simulink model "Sistemap3"  (R2026a)
settings: Solver=ode15s  StopTime=10  MaxStep=1E-2
libraries: fl_lib x14, nesl_utility x8, slpidlib x1
settings Model: Creator=Admin  LastModifiedBy=HP
settings DataIOCC: TimeSaveName=t
settings DebuggingCC: ArtificialAlgebraicLoopMsg=none  MaxConsecutiveZCsMsg=none

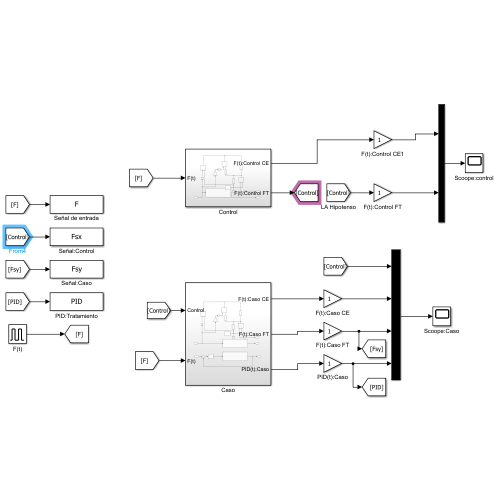
[thumbnail: Simulink's stored preview of the top-level diagram]
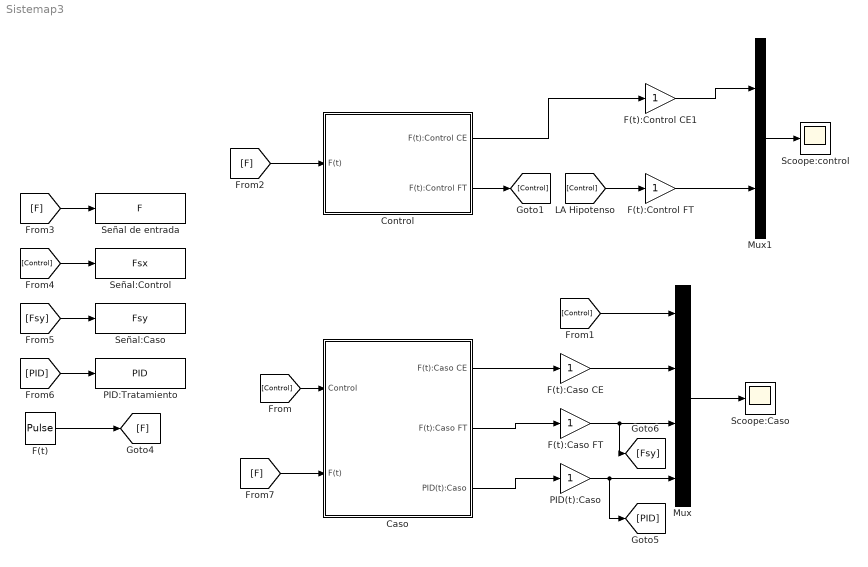
== system Sistemap3 ==
  Caso : Subsystem
  Control : Subsystem
  "F(t) " : DiscretePulseGenerator  PulseType=Time based  Period=10  PulseWidth=10  PhaseDelay=1
  F(t):Caso CE : Gain
  F(t):Caso FT : Gain
  F(t):Control CE1 : Gain
  F(t):Control FT : Gain
  Mux : Mux
  Mux1 : Mux  Inputs=2
  PID(t):Caso : Gain
  PID:Tratamiento : ToWorkspace  VariableName=PID  SampleTime=-1
  Scoope:Caso : Scope
      settings: TimeSpan=10  ActiveDisplayYMinimum=-0.21660297738034551  ActiveDisplayYMaximum=1.0433970226196547
  Scoope:control : Scope
      settings: ActiveDisplayYMinimum=-0.48996250674145203  ActiveDisplayYMaximum=1.2740374932585483
  Señal de entrada : ToWorkspace  VariableName=F  SampleTime=-1
  Señal:Caso : ToWorkspace  VariableName=Fsy  SampleTime=-1
  Señal:Control : ToWorkspace  VariableName=Fsx  SampleTime=-1
  wires:
  [Control] -> Caso/1(Control)
  [Control] -> Mux/1
  Mux/1 -> Scoope:Caso/1
  F(t):Caso CE/1 -> Mux/2
  F(t):Caso FT/1 -> [Fsy], Mux/3
  PID(t):Caso/1 -> [PID], Mux/4
  [F] -> Control/1(F(t))
  Mux1/1 -> Scoope:control/1
  Control/2(F(t):Control FT) -> [Control]
  [F] -> Señal de entrada/1
  [Control] -> Señal:Control/1
  [Fsy] -> Señal:Caso/1
  [PID] -> PID:Tratamiento/1
  "F(t) "/1 -> [F]
  [F] -> Caso/2(F(t))
  Caso/1(F(t):Caso CE) -> F(t):Caso CE/1
  Caso/2(F(t):Caso FT) -> F(t):Caso FT/1
  Caso/3(PID(t):Caso) -> PID(t):Caso/1
  [Control] -> F(t):Control FT/1
  F(t):Control FT/1 -> Mux1/2
  Control/1(F(t):Control CE) -> F(t):Control CE1/1
  F(t):Control CE1/1 -> Mux1/1

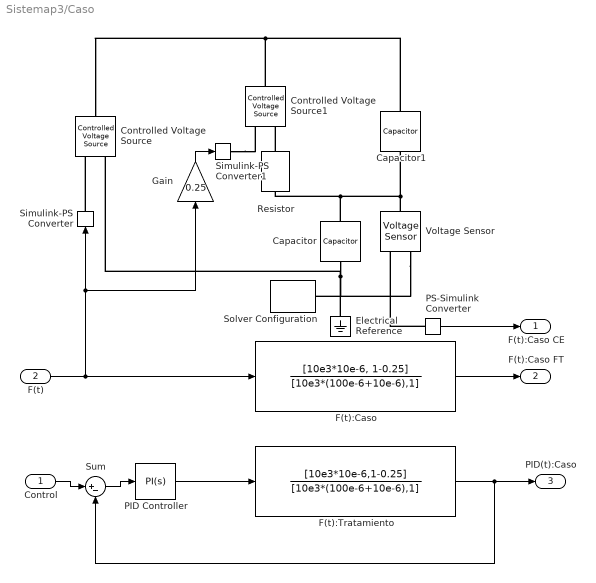
== system Sistemap3/Caso ==
  Control : Inport
  F(t) : Inport  Port=2
  Capacitor : fl_lib/Electrical/Electrical Elements/Capacitor  c=1e-6 F  r=1e-6 Ohm  g=0 1/Ohm  i_specify=off  i_priority=None  i=0 A  i_nominal_specify=off  i_nominal_value=1  i_nominal_unit=A  v_specify=off  v_priority=None  v=0 V  v_nominal_specify=off  v_nominal_value=1  v_nominal_unit=V  vc_specify=off  vc_priority=High  vc=0 V  vc_nominal_specify=off  vc_nominal_value=1  vc_nominal_unit=V
  Capacitor1 : fl_lib/Electrical/Electrical Elements/Capacitor  c=1e-6 F  r=1e-6 Ohm  g=0 1/Ohm  i_specify=off  i_priority=None  i=0 A  i_nominal_specify=off  i_nominal_value=1  i_nominal_unit=A  v_specify=off  v_priority=None  v=0 V  v_nominal_specify=off  v_nominal_value=1  v_nominal_unit=V  vc_specify=off  vc_priority=High  vc=0 V  vc_nominal_specify=off  vc_nominal_value=1  vc_nominal_unit=V
  Controlled Voltage Source : fl_lib/Electrical/Electrical Sources/Controlled Voltage Source
  Controlled Voltage Source1 : fl_lib/Electrical/Electrical Sources/Controlled Voltage Source
  Electrical Reference : fl_lib/Electrical/Electrical Elements/Electrical Reference
  F(t):Caso : TransferFcn  Numerator=[10e3*10e-6, 1-0.25]  Denominator=[10e3*(100e-6+10e-6),1]
  F(t):Tratamiento : TransferFcn  Numerator=[10e3*10e-6,1-0.25]  Denominator=[10e3*(100e-6+10e-6),1]
  Gain : Gain  Gain=0.25
  PID Controller : slpidlib/PID Controller  Controller=PI  Form=Parallel  TimeDomain=Continuous-time  UseExternalTs=off  SampleTime=-1  IntegratorMethod=Forward Euler  FilterMethod=Forward Euler  ControllerParametersSource=internal  P=0.0214581683425368  I=42291.2654382088  UseKiTs=off  D=0  UseExternalDerivativeSource=off  N=100  UseFilter=on  TunerSelectOption=Transfer Function Based (PID Tuner App)  InitialConditionSource=internal  InitialConditionForIntegrator=0  InitialConditionForFilter=0  DifferentiatorICPrevScaledInput=0  ExternalReset=none  TrackingMode=off  Kt=1  LimitOutput=off  SatLimitsSource=internal  UpperSaturationLimit=inf  LowerSaturationLimit=-inf  LinearizeAsGain=on  AntiWindupMode=none  Kb=1  LimitIntegrator=off  UpperIntegratorSaturationLimit=inf  LowerIntegratorSaturationLimit=-inf  POutMin=[]  POutMax=[]  IOutMin=[]  IOutMax=[]  DOutMin=[]  DOutMax=[]  NOutMin=[]  NOutMax=[]  SumOutMin=[]  SumOutMax=[]  SaturationOutMin=[]  SaturationOutMax=[]  PParamMin=[]  PParamMax=[]  IParamMin=[]  IParamMax=[]  DParamMin=[]  DParamMax=[]  NParamMin=[]  NParamMax=[]  KbParamMin=[]  KbParamMax=[]  KtParamMin=[]  KtParamMax=[]  KbOutMin=[]  KbOutMax=[]  KtOutMin=[]  KtOutMax=[]  IntegratorOutMin=[]  IntegratorOutMax=[]  FilterOutMin=[]  FilterOutMax=[]  SumI1OutMin=[]  SumI1OutMax=[]  SumI2OutMin=[]  SumI2OutMax=[]  SumI3OutMin=[]  SumI3OutMax=[]  SumI4OutMin=[]  SumI4OutMax=[]  SumDOutMin=[]  SumDOutMax=[]  DifferentiatorOutMin=[]  DifferentiatorOutMax=[]  FilterDiffOutCoefMin=[]  FilterDiffOutCoefMax=[]  ReciprocalOutMin=[]  ReciprocalOutMax=[]  SumDenOutMin=[]  SumDenOutMax=[]  SumNumOutMin=[]  SumNumOutMax=[]  DivideOutMin=[]  DivideOutMax=[]  UdiffTsProdOutMin=[]  UdiffTsProdOutMax=[]  NTsProdOutMin=[]  NTsProdOutMax=[]  UintegralTsProdOutMin=[]  UintegralTsProdOutMax=[]  UngainTsProdOutMin=[]  UngainTsProdOutMax=[]  ClampingZeroOutDataTypeStr=Inherit: Inherit via back propagation  ClampingZeroOutMin=[]  ClampingZeroOutMax=[]  FilterDenConstantOutDataTypeStr=Inherit: Inherit via back propagation  FilterDenConstantOutMin=[]  FilterDenConstantOutMax=[]  PCopyOutDataTypeStr=Inherit: Inherit via back propagation  PCopyOutMin=[]  PCopyOutMax=[]  NCopyOutDataTypeStr=Inherit: Inherit via back propagation  NCopyOutMin=[]  NCopyOutMax=[]  IntegratorContinuousStateAttributes=''  IntegratorStateMustResolveToSignalObject=off  IntegratorRTWStateStorageClass=Auto  FilterContinuousStateAttributes=''  FilterStateMustResolveToSignalObject=off  FilterRTWStateStorageClass=Auto  ParallelPVariant=InternalParameters  IdealPVariant=Disabled  IVariant=InternalParameters  DVariant=Disabled  IntegratorVariant=Continuous  SatVariant=Disabled  AWVariant=Passthrough  PCopyVariant=Disabled  TRVariant=Disabled  FdbkBlocksVariant=Forward  IdealPFdbkVariant=Disabled  SatFdbkVariant=Disabled  DerivativeFilterVariant=Disabled  NVariant=Disabled  NCopyVariant=Disabled_SignalSpec  FilterICVariant=Disabled  IntegratorICVariant=InternalICs  ExternalResetVariant=Disabled  TRSumVariant=Passthrough  SumFdbkVariant=Disabled  SumVariant=Sum_PI  TsampFilterVariant=InternalTs  TsampNgainVariant=Passthrough  TsampIntegralVariant=Disabled_SignalSpec  ExternalSaturationOutDataTypeStr=Inherit: Same as second input  DerivativeSourceVariant=Disabled  PreIntVariant=InternalPreInt
  PS-Simulink Converter : nesl_utility/PS-Simulink Converter  PhysicalDomain=network_engine_domain  SubClassName=ps_output  LeftPortType=input  RightPortType=output  PseudoPeriodic=off  Frequencies=[]  VectorFormat=inherit  Unit=inherit  AffineConversion=off
  Resistor : fl_lib/Electrical/Electrical Elements/Resistor  R=1 Ohm  i_specify=off  i_priority=None  i=0 A  i_nominal_specify=off  i_nominal_value=1  i_nominal_unit=A  v_specify=off  v_priority=None  v=0 V  v_nominal_specify=off  v_nominal_value=1  v_nominal_unit=V
  Simulink-PS Converter : nesl_utility/Simulink-PS Converter  PhysicalDomain=network_engine_domain  SubClassName=ps_input  LeftPortType=input  RightPortType=output  PseudoPeriodic=off  Frequencies=[]  NoiseDistribution=none  NoiseParameters=[]  Unit=1  AffineConversion=off  FilteringAndDerivatives=provide  SimscapeFilterOrder=1  InputFilterTimeConstant=0.001  UdotUserProvided=0
  Simulink-PS Converter1 : nesl_utility/Simulink-PS Converter  PhysicalDomain=network_engine_domain  SubClassName=ps_input  LeftPortType=input  RightPortType=output  PseudoPeriodic=off  Frequencies=[]  NoiseDistribution=none  NoiseParameters=[]  Unit=1  AffineConversion=off  FilteringAndDerivatives=provide  SimscapeFilterOrder=1  InputFilterTimeConstant=0.001  UdotUserProvided=0
  Solver Configuration : nesl_utility/Solver Configuration  PhysicalDomain=network_engine_domain  SubClassName=solver  LeftPortType=input  RightPortType=generic  Tones=[]  Harmonics=[]  SimulateNoise=off  Profile=off  UseLocalSampling=off  EnableSwitchedLinearOptims=on  FrequencyDomain=off  UseCCode=off  RelTol=0.001  AbsTol=0.001  MinStep=1e-09  ToWorkspace=off  RevertToSquareIcSolve=off  NumHomotopyIterations=100  PhasorMode=off  PhasorModeNumHarmonics=1  ConsistencySolver=NEWTON_XTOL_AFTER_FTOL  CanonicalOrdering=CANONICAL  OptimizeIntermediates=OPTIMIZED  IndexReductionMethod=DerivativeReplacement  DoDC=off  ResidualTolerance=1e-09  ConsistencyTolSource=GLOBAL  ConsistencyAbsTol=0.001  ConsistencyRelTol=0.001  ConsistencyTolFactor=0.001  UseLocalSolver=off  LocalSolverChoice=NE_BACKWARD_EULER_ADVANCER  ResolveIndetEquations=on  FunctionEvalNumThread=1  LocalSolverSampleTime=0.001  DoFixedCost=off  MaxNonlinIter=3  MaxModeIter=2  ComputeImpulses=off  ImpulseIterations=2  LinearAlgebra=auto  LinearAlgebraNumThread=0  EquationFormulation=NE_TIME_EF  DelaysMemoryBudget=1024  AutomaticFiltering=on  FilteringTimeConstant=0.001  PartitionStorageMethod=AS_NEEDED  PartitionMemoryBudget=1024  PartitionMethod=ROBUST  MultibodyUseLocalSolver=off  MultibodyLocalSolverChoice=ODE1  MultibodyLocalSolverSampleTime=0.001
  Sum : Sum  Inputs=|+-
  Voltage Sensor : fl_lib/Electrical/Electrical Sensors/Voltage Sensor
  F(t):Caso CE : Outport
  F(t):Caso FT : Outport  Port=2
  PID(t):Caso : Outport  Port=3
  wires:
  F(t)/1 -> F(t):Caso/1, Gain/1, Simulink-PS Converter/1
  F(t):Caso/1 -> F(t):Caso FT/1
  PS-Simulink Converter/1 -> F(t):Caso CE/1
  Gain/1 -> Simulink-PS Converter1/1
  PID Controller/1 -> F(t):Tratamiento/1
  Control/1 -> Sum/1
  Sum/1 -> PID Controller/1
  F(t):Tratamiento/1 -> Sum/2, PID(t):Caso/1
  connections:
  Capacitor/RConn1 -- Electrical Reference/LConn1 -- Voltage Sensor/RConn2 -- Solver Configuration/RConn1 -- Controlled Voltage Source/RConn2
  Voltage Sensor/LConn1 -- Resistor/RConn1 -- Capacitor/LConn1 -- Capacitor1/RConn1
  Controlled Voltage Source1/LConn1 -- Capacitor1/LConn1 -- Controlled Voltage Source/LConn1
  Resistor/LConn1 -- Controlled Voltage Source1/RConn2
  PS-Simulink Converter/LConn1 -- Voltage Sensor/RConn1
  Simulink-PS Converter1/RConn1 -- Controlled Voltage Source1/RConn1
  Simulink-PS Converter/RConn1 -- Controlled Voltage Source/RConn1

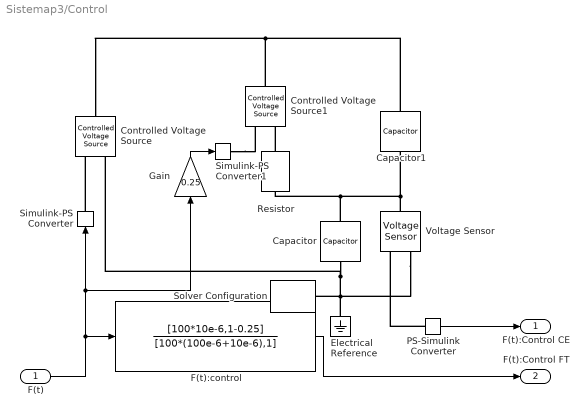
== system Sistemap3/Control ==
  F(t) : Inport
  Capacitor : fl_lib/Electrical/Electrical Elements/Capacitor  c=1e-6 F  r=1e-6 Ohm  g=0 1/Ohm  i_specify=off  i_priority=None  i=0 A  i_nominal_specify=off  i_nominal_value=1  i_nominal_unit=A  v_specify=off  v_priority=None  v=0 V  v_nominal_specify=off  v_nominal_value=1  v_nominal_unit=V  vc_specify=off  vc_priority=High  vc=0 V  vc_nominal_specify=off  vc_nominal_value=1  vc_nominal_unit=V
  Capacitor1 : fl_lib/Electrical/Electrical Elements/Capacitor  c=1e-6 F  r=1e-6 Ohm  g=0 1/Ohm  i_specify=off  i_priority=None  i=0 A  i_nominal_specify=off  i_nominal_value=1  i_nominal_unit=A  v_specify=off  v_priority=None  v=0 V  v_nominal_specify=off  v_nominal_value=1  v_nominal_unit=V  vc_specify=off  vc_priority=High  vc=0 V  vc_nominal_specify=off  vc_nominal_value=1  vc_nominal_unit=V
  Controlled Voltage Source : fl_lib/Electrical/Electrical Sources/Controlled Voltage Source
  Controlled Voltage Source1 : fl_lib/Electrical/Electrical Sources/Controlled Voltage Source
  Electrical Reference : fl_lib/Electrical/Electrical Elements/Electrical Reference
  F(t):control : TransferFcn  Numerator=[100*10e-6,1-0.25]  Denominator=[100*(100e-6+10e-6),1]
  Gain : Gain  Gain=0.25
  PS-Simulink Converter : nesl_utility/PS-Simulink Converter  PhysicalDomain=network_engine_domain  SubClassName=ps_output  LeftPortType=input  RightPortType=output  PseudoPeriodic=off  Frequencies=[]  VectorFormat=inherit  Unit=inherit  AffineConversion=off
  Resistor : fl_lib/Electrical/Electrical Elements/Resistor  R=1 Ohm  i_specify=off  i_priority=None  i=0 A  i_nominal_specify=off  i_nominal_value=1  i_nominal_unit=A  v_specify=off  v_priority=None  v=0 V  v_nominal_specify=off  v_nominal_value=1  v_nominal_unit=V
  Simulink-PS Converter : nesl_utility/Simulink-PS Converter  PhysicalDomain=network_engine_domain  SubClassName=ps_input  LeftPortType=input  RightPortType=output  PseudoPeriodic=off  Frequencies=[]  NoiseDistribution=none  NoiseParameters=[]  Unit=1  AffineConversion=off  FilteringAndDerivatives=provide  SimscapeFilterOrder=1  InputFilterTimeConstant=0.001  UdotUserProvided=0
  Simulink-PS Converter1 : nesl_utility/Simulink-PS Converter  PhysicalDomain=network_engine_domain  SubClassName=ps_input  LeftPortType=input  RightPortType=output  PseudoPeriodic=off  Frequencies=[]  NoiseDistribution=none  NoiseParameters=[]  Unit=1  AffineConversion=off  FilteringAndDerivatives=provide  SimscapeFilterOrder=1  InputFilterTimeConstant=0.001  UdotUserProvided=0
  Solver Configuration : nesl_utility/Solver Configuration  PhysicalDomain=network_engine_domain  SubClassName=solver  LeftPortType=input  RightPortType=generic  Tones=[]  Harmonics=[]  SimulateNoise=off  Profile=off  UseLocalSampling=off  EnableSwitchedLinearOptims=on  FrequencyDomain=off  UseCCode=off  RelTol=0.001  AbsTol=0.001  MinStep=1e-09  ToWorkspace=off  RevertToSquareIcSolve=off  NumHomotopyIterations=100  PhasorMode=off  PhasorModeNumHarmonics=1  ConsistencySolver=NEWTON_XTOL_AFTER_FTOL  CanonicalOrdering=CANONICAL  OptimizeIntermediates=OPTIMIZED  IndexReductionMethod=DerivativeReplacement  DoDC=off  ResidualTolerance=1e-09  ConsistencyTolSource=GLOBAL  ConsistencyAbsTol=0.001  ConsistencyRelTol=0.001  ConsistencyTolFactor=0.001  UseLocalSolver=off  LocalSolverChoice=NE_BACKWARD_EULER_ADVANCER  ResolveIndetEquations=on  FunctionEvalNumThread=1  LocalSolverSampleTime=0.001  DoFixedCost=off  MaxNonlinIter=3  MaxModeIter=2  ComputeImpulses=off  ImpulseIterations=2  LinearAlgebra=auto  LinearAlgebraNumThread=0  EquationFormulation=NE_TIME_EF  DelaysMemoryBudget=1024  AutomaticFiltering=on  FilteringTimeConstant=0.001  PartitionStorageMethod=AS_NEEDED  PartitionMemoryBudget=1024  PartitionMethod=ROBUST  MultibodyUseLocalSolver=off  MultibodyLocalSolverChoice=ODE1  MultibodyLocalSolverSampleTime=0.001
  Voltage Sensor : fl_lib/Electrical/Electrical Sensors/Voltage Sensor
  F(t):Control CE : Outport
  F(t):Control FT : Outport  Port=2
  wires:
  F(t):control/1 -> F(t):Control FT/1
  Gain/1 -> Simulink-PS Converter1/1
  F(t)/1 -> F(t):control/1, Gain/1, Simulink-PS Converter/1
  PS-Simulink Converter/1 -> F(t):Control CE/1
  connections:
  Controlled Voltage Source1/LConn1 -- Capacitor1/LConn1 -- Controlled Voltage Source/LConn1
  Resistor/LConn1 -- Controlled Voltage Source1/RConn2
  Voltage Sensor/LConn1 -- Resistor/RConn1 -- Capacitor/LConn1 -- Capacitor1/RConn1
  Voltage Sensor/RConn2 -- Controlled Voltage Source/RConn2 -- Capacitor/RConn1 -- Electrical Reference/LConn1 -- Solver Configuration/RConn1
  Simulink-PS Converter/RConn1 -- Controlled Voltage Source/RConn1
  Simulink-PS Converter1/RConn1 -- Controlled Voltage Source1/RConn1
  PS-Simulink Converter/LConn1 -- Voltage Sensor/RConn1
